simulink library "StateMachine"  (R2023b)
settings: Solver=VariableStepAuto  StartTime=0.0  StopTime=10.0  RelTol=1e-3
values from neighbouring files (symbols this model uses):
  toKukaEtherCatStruct = Simulink.Bus.createMATLABStruct('ToKukaEtherCat')    [initStateMachineParameters.m]
undefined symbols (not defined in the file or in its folder): SM_STATES, Ts
settings Model: Creator=muralikarnam  LastModifiedBy=User
settings SolverCC: AlgebraicLoopSolver=TrustRegion
settings DataIOCC: ReturnWorkspaceOutputs=off
settings DebuggingCC: UnconnectedInputMsg=warning  UnconnectedOutputMsg=warning  UnconnectedLineMsg=warning  ArithmeticOperatorsInVariantConditions=warning
settings ModelReferenceCC: EnableRefExpFcnMdlSchedulingChecks=on
settings SFSimCC: SimUseLocalCustomCode=off  CustomCodeUndefinedFunction=UseInterfaceOnly
settings RTWCC: RTWUseLocalCustomCode=off

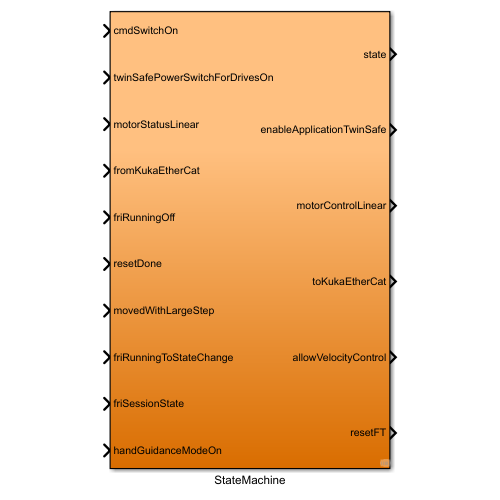
[thumbnail: Simulink's stored preview of the top-level diagram]
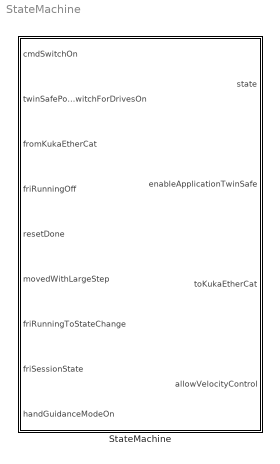
== system StateMachine ==
  StateMachine : Subsystem

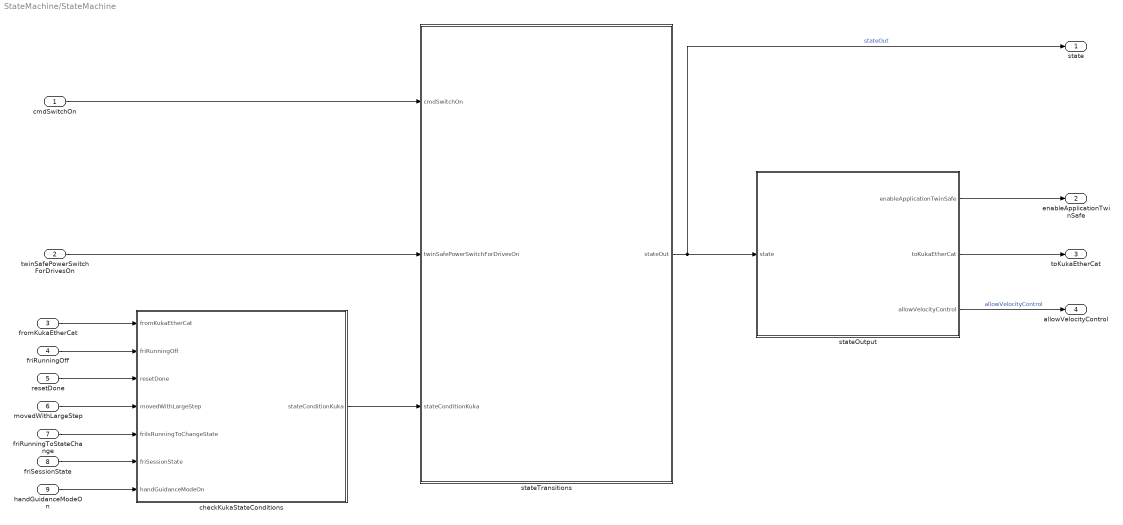
== system StateMachine/StateMachine ==
  cmdSwitchOn : Inport  OutDataTypeStr=boolean  PortDimensions=1
  twinSafePowerSwitchForDrivesOn : Inport  Port=2  OutDataTypeStr=boolean  PortDimensions=1  SampleTime=0
  fromKukaEtherCat : Inport  Port=3  OutDataTypeStr=Bus: FromKukaEtherCat
  friRunningOff : Inport  Port=4  OutDataTypeStr=boolean
  resetDone : Inport  Port=5  OutDataTypeStr=boolean  PortDimensions=1
  movedWithLargeStep : Inport  Port=6  OutDataTypeStr=boolean  PortDimensions=1
  friRunningToStateChange : Inport  Port=7  OutDataTypeStr=boolean
  friSessionState : Inport  Port=8  OutDataTypeStr=uint8  PortDimensions=1
  handGuidanceModeOn : Inport  Port=9  OutDataTypeStr=boolean  PortDimensions=1
  checkKukaStateConditions : MATLAB Function  TreatAsAtomicUnit=on
  stateOutput : MATLAB Function  TreatAsAtomicUnit=on
  stateTransitions : MATLAB Function  TreatAsAtomicUnit=on
  state : Outport  OutDataTypeStr=double  PortDimensions=1  SampleTime=0  VectorParamsAs1DForOutWhenUnconnected=off
  enableApplicationTwinSafe : Outport  Port=2  OutDataTypeStr=boolean  PortDimensions=1  SampleTime=0  VectorParamsAs1DForOutWhenUnconnected=off
  toKukaEtherCat : Outport  Port=3  OutDataTypeStr=Bus: ToKukaEtherCat  VectorParamsAs1DForOutWhenUnconnected=off
  allowVelocityControl : Outport  Port=4  OutDataTypeStr=boolean  PortDimensions=1  SampleTime=0  VectorParamsAs1DForOutWhenUnconnected=off
  wires:
  friRunningToStateChange/1 -> checkKukaStateConditions/5(friIsRunningToChangeState)
  movedWithLargeStep/1 -> checkKukaStateConditions/4(movedWithLargeStep)
  stateOutput/2(toKukaEtherCat) -> toKukaEtherCat/1
  resetDone/1 -> checkKukaStateConditions/3(resetDone)
  checkKukaStateConditions/1(stateConditionKuka) -> stateTransitions/3(stateConditionKuka)
  friRunningOff/1 -> checkKukaStateConditions/2(friRunningOff)
  fromKukaEtherCat/1 -> checkKukaStateConditions/1(fromKukaEtherCat)
  stateOutput/1(enableApplicationTwinSafe) -> enableApplicationTwinSafe/1
  stateOutput/3(allowVelocityControl) -> allowVelocityControl/1  "allowVelocityControl"
  cmdSwitchOn/1 -> stateTransitions/1(cmdSwitchOn)
  twinSafePowerSwitchForDrivesOn/1 -> stateTransitions/2(twinSafePowerSwitchForDrivesOn)
  stateTransitions/1(stateOut) -> stateOutput/1(state), state/1  "stateOut"
  friSessionState/1 -> checkKukaStateConditions/6(friSessionState)
  handGuidanceModeOn/1 -> checkKukaStateConditions/7(handGuidanceModeOn)

== matlab function StateMachine/stateOutput ==
  data: enableApplicationTwinSafe output boolean size=1; state input double size=1; toKukaEtherCat output Bus: ToKukaEtherCat; allowVelocityControl output boolean size=1; SM_STATES parameter; toKukaEtherCatStruct parameter Bus: ToKukaEtherCat
%#codegen
function [enableApplicationTwinSafe, toKukaEtherCat, allowVelocityControl]=stateOutputs(state, SM_STATES, toKukaEtherCatStruct)
%2019-05-24 Nicolas Gerig
%2020-03-26 Murali Karnam
%2024-09-27 Ruben Martin Rodriguez

%% default outputs
enableApplicationTwinSafe = false;
allowVelocityControl = false;

kukaAppEnable = false;
kukaAppStart = false;
kukaShouldServerRun = false;
kukaShouldFriRun = false;
kukaShouldHoldPosition = false;
kukaResetPosition = false;
kukaLargeJointStep = false;
kukaResetPositionDoneFromSM = false;

toKukaEtherCat = toKukaEtherCatStruct;



%% switch outputs based on state
switch state
    
    case SM_STATES.INIT
        
    case  SM_STATES.RESETTING_MOTOR_DRIVES
        
    case  SM_STATES.SWITCHING_ON_AND_WAIT_FOR_TWINSAFE_POWER
        
        enableApplicationTwinSafe = true;
        
    case  SM_STATES.KUKA_ENABLING_APP
        
        enableApplicationTwinSafe = true;
        kukaAppEnable = true;
        kukaShouldServerRun = true;
        
        
    case  SM_STATES.KUKA_STARTING_APP
        
        enableApplicationTwinSafe = true;
        kukaAppEnable = true;
        kukaShouldServerRun = true;
        kukaAppStart = true;
        
    case  SM_STATES.KUKA_STARTING_FRI
        
        enableApplicationTwinSafe = true;
        
        kukaAppEnable = true;
        kukaAppStart = true;
        kukaShouldServerRun = true;
        kukaShouldFriRun = true;
        
        
    case  SM_STATES.RESETTING_POSITIONS
        
        enableApplicationTwinSafe = true;
        
        kukaAppEnable = true;
        kukaShouldServerRun = true;
        kukaShouldFriRun = true;
        kukaResetPosition = true;
    
    case  SM_STATES.ENABLE_KUKA_HANDGUIDANCE
        
        enableApplicationTwinSafe = true;
        
        kukaAppEnable = true;
        kukaShouldServerRun = true;
        kukaShouldFriRun = true;
        kukaResetPosition = true;
        
    case  SM_STATES.ENABLING_OPERATION
        
        enableApplicationTwinSafe = true;
        
        kukaAppEnable = true;
        kukaShouldServerRun = true;
        kukaShouldFriRun = true;
        kukaShouldHoldPosition = true;
        kukaResetPositionDoneFromSM = true;
        
    case  SM_STATES.OPERATION_WITH_LARGEJOINTSTEPS
        
        enableApplicationTwinSafe = true;
        allowVelocityControl = true;
        
        kukaAppEnable = true;
        kukaShouldServerRun = true;
        kukaShouldFriRun = true;
        kukaShouldHoldPosition = true;
        kukaLargeJointStep = true;
        kukaResetPositionDoneFromSM = true;
        
    case  SM_STATES.OPERATION
        
        enableApplicationTwinSafe = true;
        allowVelocityControl = true;
        
        kukaAppEnable = true;
        kukaShouldServerRun = true;
        kukaShouldFriRun = true;
        kukaShouldHoldPosition = true;
        kukaResetPositionDoneFromSM = true;
        
    case  SM_STATES.ERROR
        
end

toKukaEtherCat.extCtrlCmdWord = kukaAutExt_cmdWord(kukaAppEnable, kukaAppStart);
toKukaEtherCat.appCtrlCmdWord= kukaFri_cmdWord(kukaShouldServerRun, kukaShouldFriRun, kukaShouldHoldPosition);
toKukaEtherCat.resetPosition = kukaResetPosition;
toKukaEtherCat.largeJointStep = kukaLargeJointStep;
toKukaEtherCat.resetPositionDoneFromSM = kukaResetPositionDoneFromSM;


%% used motor control words AX5XXX
% https://download.beckhoff.com/download/Document/motion/ax5000-s-idn-descriptions_de.pdf

    function kukaCmdWord = kukaAutExt_cmdWord(kukaAppEnable, kukaAppStart)
        kukaCmdWord = bin2dec('00000000 00000000 00000000 00000000');
        
        if(kukaAppEnable)
            kukaCmdWord = bitset(kukaCmdWord, 1);
        end
        
        if(kukaAppStart)
            kukaCmdWord = bitset(kukaCmdWord, 9);
        end
        
        kukaCmdWord = uint32(kukaCmdWord);
    end

    function kukaCmdWord = kukaFri_cmdWord(kukaShouldServerRun, kukaShouldFriRun, kukaShouldHoldPosition)
        kukaCmdWord = bin2dec('00000000 00000000 00000000 00000000');
        
        if(kukaShouldServerRun)
            kukaCmdWord = bitset(kukaCmdWord, 1);
        end
        
        if(kukaShouldFriRun)
            kukaCmdWord = bitset(kukaCmdWord, 9);
        end
        
        if(kukaShouldHoldPosition)
            kukaCmdWord = bitset(kukaCmdWord, 17);
        end
        
        kukaCmdWord = uint32(kukaCmdWord);
    end

end

== matlab function StateMachine/stateTransitions ==
  data: cmdSwitchOn input boolean size=1; twinSafePowerSwitchForDrivesOn input boolean size=1; stateConditionKuka input Bus: StateConditionKuka; stateOut output double size=1; Ts parameter; SM_STATES parameter
%#codegen
function stateOut  = stateTransitions(cmdSwitchOn, twinSafePowerSwitchForDrivesOn, stateConditionKuka, Ts, SM_STATES)
%2019-05-24 Nicolas Gerig 
%2020-03-26 Murali Karnam
%2024-09-27 Ruben Martin Rodriguez

%% persistent state variables
persistent state timer
if isempty(state) %initialization (entry)
    state = SM_STATES.INIT;
    timer = 0;
end

%% update time in state (will be reset in transitions)
timer=timer+Ts;

%% check for state transitions
switch state
    
    case SM_STATES.INIT %0
        
        if (~cmdSwitchOn) % if not commanded to switch on reenter INIT
            transitionTo(SM_STATES.INIT);%basically, just reset timer
        elseif (timer>0.1)
            transitionTo(SM_STATES.RESETTING_MOTOR_DRIVES);
        end
                        
    case SM_STATES.RESETTING_MOTOR_DRIVES %1
        
        if (~cmdSwitchOn)
            transitionTo(SM_STATES.ERROR);
        elseif (timer>0.5)
            transitionTo(SM_STATES.SWITCHING_ON_AND_WAIT_FOR_TWINSAFE_POWER);
        end
      
    case  SM_STATES.SWITCHING_ON_AND_WAIT_FOR_TWINSAFE_POWER %2
        
        if (~cmdSwitchOn)
            transitionTo(SM_STATES.ERROR);
        elseif (twinSafePowerSwitchForDrivesOn && ~stateConditionKuka.stationError)
            transitionTo(SM_STATES.KUKA_ENABLING_APP);
        elseif (~twinSafePowerSwitchForDrivesOn)
            transitionTo(SM_STATES.SWITCHING_ON_AND_WAIT_FOR_TWINSAFE_POWER);
        elseif ((timer>5))
            transitionTo(SM_STATES.ERROR);
        end
        
    case SM_STATES.KUKA_ENABLING_APP %3
        
        if (~cmdSwitchOn || stateConditionKuka.stationError || ~twinSafePowerSwitchForDrivesOn)
            transitionTo(SM_STATES.ERROR);
        elseif(stateConditionKuka.autExt_Active && stateConditionKuka.autExt_AppReadyToStart && timer>0.1)
            transitionTo(SM_STATES.KUKA_STARTING_APP);
        elseif(~stateConditionKuka.autExt_Active && timer>0.1)
            transitionTo(SM_STATES.KUKA_STARTING_APP); 
        elseif(timer>5)
            transitionTo(SM_STATES.ERROR);
        end

    case SM_STATES.KUKA_STARTING_APP %4
        
        if (~cmdSwitchOn || stateConditionKuka.stationError || ~twinSafePowerSwitchForDrivesOn)
            transitionTo(SM_STATES.ERROR);
        elseif(stateConditionKuka.autExt_Active  && ~stateConditionKuka.autExt_AppReadyToStart)
            transitionTo(SM_STATES.KUKA_STARTING_APP); % Reset timer and wait for kuka to start the App
        elseif(stateConditionKuka.autExt_Active  && stateConditionKuka.autExt_AppReadyToStart)
            transitionTo(SM_STATES.KUKA_STARTING_FRI); 
        elseif(~stateConditionKuka.autExt_Active)
            transitionTo(SM_STATES.KUKA_STARTING_FRI);
        elseif(timer>5)
            transitionTo(SM_STATES.ERROR);
        end
        

    case SM_STATES.KUKA_STARTING_FRI %5
        
        if (~cmdSwitchOn || stateConditionKuka.stationError || ~twinSafePowerSwitchForDrivesOn)
            transitionTo(SM_STATES.ERROR);
        elseif(stateConditionKuka.default_AppError)
            transitionTo(SM_STATES.ERROR);
        elseif(~stateConditionKuka.friRunningOff && stateConditionKuka.friIsRunningToChangeState)
                transitionTo(SM_STATES.RESETTING_POSITIONS);
%         elseif(~stateConditionKuka.friRunningOff && stateConditionKuka.friIsRunningToChangeState)
%             if(stateConditionKuka.handGuidanceModeOn)
%                 transitionTo(SM_STATES.KUKA_STARTING_FRI); %Wait here for hand guidance mode from Kuka
%             else
%                 transitionTo(SM_STATES.RESETTING_POSITIONS);
%             end
        elseif(~stateConditionKuka.autExt_Active  && stateConditionKuka.friRunningOff && stateConditionKuka.friIsRunningToChangeState)
            transitionTo(SM_STATES.KUKA_STARTING_FRI); % Reset timer and wait for user to start the app
        elseif(timer>5)
            transitionTo(SM_STATES.ERROR);
        end
        
    case SM_STATES.RESETTING_POSITIONS %6
        
        if (~cmdSwitchOn || stateConditionKuka.stationError || ~twinSafePowerSwitchForDrivesOn)
            transitionTo(SM_STATES.ERROR);
        elseif(stateConditionKuka.default_AppError || stateConditionKuka.friRunningOff)
            transitionTo(SM_STATES.ERROR);
        elseif(stateConditionKuka.resetDone && stateConditionKuka.friIsRunningToChangeState)
            if(stateConditionKuka.handGuidanceModeOn)
                transitionTo(SM_STATES.ENABLE_KUKA_HANDGUIDANCE); %Wait here for hand guidance mode from Kuka
            else
                transitionTo(SM_STATES.ENABLING_OPERATION);
            end
%             transitionTo(SM_STATES.ENABLING_OPERATION);
        elseif(timer>5)
            transitionTo(SM_STATES.ERROR);
        end
        
    case SM_STATES.ENABLE_KUKA_HANDGUIDANCE %65
        
        if (~cmdSwitchOn || stateConditionKuka.stationError || ~twinSafePowerSwitchForDrivesOn)
            transitionTo(SM_STATES.ERROR);
        elseif(stateConditionKuka.default_AppError || stateConditionKuka.friRunningOff)
            transitionTo(SM_STATES.ERROR);
        elseif(stateConditionKuka.handGuidanceModeOn)
            transitionTo(SM_STATES.ENABLE_KUKA_HANDGUIDANCE);
        elseif(~stateConditionKuka.handGuidanceModeOn && stateConditionKuka.friIsRunningToChangeState)
            transitionTo(SM_STATES.ENABLING_OPERATION);
        elseif(timer>5)
            transitionTo(SM_STATES.ERROR);
        end        
        
    case SM_STATES.ENABLING_OPERATION %7
        
        if (~cmdSwitchOn || stateConditionKuka.stationError  || ~twinSafePowerSwitchForDrivesOn)
            transitionTo(SM_STATES.ERROR);
        elseif(stateConditionKuka.default_AppError || stateConditionKuka.friRunningOff )
            transitionTo(SM_STATES.ERROR);
        elseif (~stateConditionKuka.movedWithLargeStep && timer > 1.0)
            transitionTo(SM_STATES.OPERATION_WITH_LARGEJOINTSTEPS);
        elseif (stateConditionKuka.movedWithLargeStep && timer > 1.0)
            transitionTo(SM_STATES.OPERATION);
        elseif (timer>5)
            transitionTo(SM_STATES.ERROR);
        end
        
    case SM_STATES.OPERATION_WITH_LARGEJOINTSTEPS %8
        
        if (~cmdSwitchOn || stateConditionKuka.stationError || ~twinSafePowerSwitchForDrivesOn)
            transitionTo(SM_STATES.ERROR);
        elseif(stateConditionKuka.default_AppError || stateConditionKuka.friRunningOff || stateConditionKuka.friSessionState < 3)
            transitionTo(SM_STATES.ERROR);
        elseif(stateConditionKuka.movedWithLargeStep && timer > 0.025)
            transitionTo(SM_STATES.OPERATION); %wait here
        elseif(~stateConditionKuka.movedWithLargeStep)
            transitionTo(SM_STATES.OPERATION_WITH_LARGEJOINTSTEPS); %resetting the timer and waiting here. 
        end
        
    case SM_STATES.OPERATION %9
        
        if (~cmdSwitchOn || stateConditionKuka.stationError || ~twinSafePowerSwitchForDrivesOn)
            transitionTo(SM_STATES.ERROR);
        elseif(stateConditionKuka.default_AppError || stateConditionKuka.friRunningOff || stateConditionKuka.friSessionState < 3)
            transitionTo(SM_STATES.ERROR);
        end
        
    case SM_STATES.ERROR %10
        
        if timer>1
            transitionTo(SM_STATES.INIT);
        end
end

%% outputs:
stateOut=state;

%% transition helper functions
    function transitionTo(newState)
        state = newState;
        timer = 0;
    end

end

== matlab function StateMachine/checkKukaStateConditions ==
  data: fromKukaEtherCat input Bus: FromKukaEtherCat size=1; stateConditionKuka output Bus: StateConditionKuka size=1; friRunningOff input boolean size=1; resetDone input boolean size=1; movedWithLargeStep input; friIsRunningToChangeState input; friSessionState input; handGuidanceModeOn input boolean size=1
%#codegen
function stateConditionKuka = checkKukaStateConditions(fromKukaEtherCat, friRunningOff, resetDone, movedWithLargeStep,  friIsRunningToChangeState, friSessionState, handGuidanceModeOn)
%2020-03-26 Murali Karnam

%% outputs:
stateConditionKuka.autExt_Active= checkKuka_AutExt_Active( fromKukaEtherCat.extCtrlStatusWord );
stateConditionKuka.autExt_AppReadyToStart = checkKuka_AutExt_AppReadyToStart( fromKukaEtherCat.extCtrlStatusWord );
stateConditionKuka.default_AppError = checkKuka_Default_AppError( fromKukaEtherCat.extCtrlStatusWord );
stateConditionKuka.stationError = checkKuka_StationError( fromKukaEtherCat.extCtrlStatusWord );
%stateConditionKuka.serverRunningOn = checkKuka_ServerStatus( fromKukaEtherCat.serverStatusWord );
stateConditionKuka.friRunningOff = friRunningOff;
stateConditionKuka.resetDone = resetDone;
stateConditionKuka.movedWithLargeStep = movedWithLargeStep;
stateConditionKuka.friIsRunningToChangeState = friIsRunningToChangeState;
stateConditionKuka.friSessionState = friSessionState;
stateConditionKuka.handGuidanceModeOn = handGuidanceModeOn;



%% Status word checks Kuka:
%These are connections made in WorkVisual on the Kuka Side by packing 4
%booleans into one uint32

	function bResult = checkKuka_AutExt_Active(kukaStatusword)
        %bit-1 
        bResult = ( checkIfBit_TRUE( kukaStatusword, 0 ) );
    end

	function bResult = checkKuka_AutExt_AppReadyToStart(kukaStatusword)
        %bit-8 
        bResult = ( checkIfBit_TRUE( kukaStatusword, 8 ) );
    end

	function bResult = checkKuka_Default_AppError(kukaStatusword)
        %bit-16 
        bResult = ( checkIfBit_TRUE( kukaStatusword, 16 ) );
    end

	function bResult = checkKuka_StationError(kukaStatusword)
        %bit-24 
        bResult = ( checkIfBit_TRUE( kukaStatusword, 24 ) );
    end

% 	function bResult = checkKuka_ServerStatus(kukaStatusword)
%         %bit-1 
%         bResult = ( checkIfBit_TRUE( kukaStatusword, 0 ) );
%     end


%% helper functions
    function bResult = checkIfBit_TRUE(value, bitNumber)
        bResult = ( bitand(value,2^bitNumber) == 2^bitNumber );
    end

    function bResult = checkIfBit_FALSE(value, bitNumber)
        bResult = ( bitand(value,2^bitNumber) == 0 );
    end

end
